simulink model "CombinedExperiment"  (R2020a)
settings: Solver=FixedStepAuto  StartTime=0.0  StopTime=tsim  FixedStep=baseRate  RelTol=1e-3  EnableMultiTasking=on
values from neighbouring files (symbols this model uses):
  baseRate = 0.1    [Run_Initializer.m]
  drop_states_BLACK = [1.36947387695313,1.22175756835938,-0.0161599479615688]    [Run_Initializer.m]
  drop_states_BLUE = [ xLength/2+0.9; yLength/2+0.5; 0]    [Run_Initializer.m]
  drop_states_RED = [ xLength/2+1.1; yLength/2; pi]    [Run_Initializer.m]
  F_thrusters_BLACK = 0.25.*ones(8,1)    [Run_Initializer.m]
  F_thrusters_BLUE = 0.25.*ones(8,1)    [Run_Initializer.m]
  F_thrusters_RED = 0.25.*ones(8,1)    [Run_Initializer.m]
  home_states_BLACK = [ xLength/2; yLength/2; 0]    [Run_Initializer.m]
  home_states_BLUE = [ xLength/2-0.9; yLength/2+0.5; 0]    [Run_Initializer.m]
  home_states_RED = [ xLength/2+1.1; yLength/2; pi]    [Run_Initializer.m]
  init_states_BLACK = [ xLength/2; yLength/2; 0]    [Run_Initializer.m]
  init_states_BLUE = [ xLength/2+0.9; yLength/2+0.5; 0]    [Run_Initializer.m]
  init_states_RED = [ xLength/2+1.1; yLength/2; pi]    [Run_Initializer.m]
  Kd_tb = 0.4    [Run_Initializer.m]
  Kd_tblue = 0.4    [Run_Initializer.m]
  Kd_tr = 0.4    [Run_Initializer.m]
  Kd_xb = 5    [Run_Initializer.m]
  Kd_xblue = 5    [Run_Initializer.m]
  Kd_xr = 5    [Run_Initializer.m]
  Kd_yb = 5    [Run_Initializer.m]
  Kd_yblue = 5    [Run_Initializer.m]
  Kd_yr = 5    [Run_Initializer.m]
  Kp_tb = 0.1    [Run_Initializer.m]
  Kp_tblue = 0.1    [Run_Initializer.m]
  Kp_tr = 0.1    [Run_Initializer.m]
  Kp_xb = 2    [Run_Initializer.m]
  Kp_xblue = 2    [Run_Initializer.m]
  Kp_xr = 2    [Run_Initializer.m]
  Kp_yb = 2    [Run_Initializer.m]
  Kp_yblue = 2    [Run_Initializer.m]
  Kp_yr = 2    [Run_Initializer.m]
  noise_variance_BLACK = 0    [Run_Initializer.m]
  noise_variance_BLUE = 0    [Run_Initializer.m]
  noise_variance_RED = 0    [Run_Initializer.m]
  Phase0_End = Phase0_Duration    (= 10)    [Run_Initializer.m]
  Phase1_End = Phase0_Duration + Phase1_Duration    (= 15)    [Run_Initializer.m]
  Phase2_End = Phase0_Duration + Phase1_Duration +                                   Phase2_Duration    (= 40)    [Run_Initializer.m]
  Phase3_End = Phase0_Duration + Phase1_Duration +                                   Phase2_Duration + Phase3_Duration    (= 117)    [Run_Initializer.m]
  Phase3_SubPhase1_End = Phase2_End + Phase3_SubPhase1_Duration    (= 41)    [Run_Initializer.m]
  Phase3_SubPhase2_End = Phase2_End + Phase3_SubPhase1_Duration +                                   Phase3_SubPhase2_Duration    (= 42)    [Run_Initializer.m]
  Phase3_SubPhase3_End = Phase2_End + Phase3_SubPhase1_Duration +                                   Phase3_SubPhase2_Duration +                                  Phase3_SubPhase3_Duration    (= 72)    [Run_Initializer.m]
  Phase3_SubPhase4_End = Phase2_End + Phase3_SubPhase1_Duration +                                   Phase3_SubPhase2_Duration +                                  Phase3_SubPhase3_Duration +                                  Phase3_SubPhase4_Duration    [Run_Initializer.m]
  Phase4_End = Phase0_Duration + Phase1_Duration +                                   Phase2_Duration + Phase3_Duration +                                   Phase4_Duration    (= 137)    [Run_Initializer.m]
  Phase5_End = Phase0_Duration + Phase1_Duration +                                   Phase2_Duration + Phase3_Duration +                                   Phase4_Duration + Phase5_Duration    (= 142)    [Run_Initializer.m]
  serverRate = 0.2    [Run_Initializer.m]
  thruster_dist2CG_BLACK = [83.42;-52.58;55.94;-60.05;54.08;-53.92;77.06;-55.94]    [Run_Initializer.m]
  thruster_dist2CG_BLUE = [83.42;-52.58;55.94;-60.05;54.08;-53.92;77.06;-55.94]    [Run_Initializer.m]
  thruster_dist2CG_RED = [49.92;-78.08;70.46;-63.54;81.08;-50.42;57.44;-75.96]    [Run_Initializer.m]
  xLength = 3.51155    [Run_Initializer.m]
  yLength = 2.41935    [Run_Initializer.m]
undefined symbols (not defined in the file or in its folder): DiscIntNeverNeededParam, platformSelection, simMode, WhoAmI
libraries: dspstat3 x18, raspberrypiBasiclib x10, dspsigops x9, embdlinuxlib x8, simulink x8, MainLibrary x5, mspfiltlib x3, dsparch4 x3, dspswit3 x2, sensehatlib x1
(part 3 of 9)

== system CombinedExperiment/Phase #2: Move to Initial Position/Change BLACK Behavior ==
  note: Additional Blocks
  note: PD Control Law - BLACK
  note: Additional blocks are stored here.
  note: A simple PD control law is used here to command the platform to it's initial position, as defined in the initializer.
  Action Port : ActionPort  ActionPortLabel=if(u1 == 2 | u2 == 1)
  BLACK_Fx : DataStoreWrite  DataStoreName=BLACK_Fx
  BLACK_Fy : DataStoreWrite  DataStoreName=BLACK_Fy
  BLACK_Px : DataStoreRead  DataStoreName=BLACK_Px
  "BLACK_Py " : DataStoreRead  DataStoreName=BLACK_Py
  BLACK_Rz : DataStoreRead  DataStoreName=BLACK_Rz
  BLACK_Tz : DataStoreWrite  DataStoreName=BLACK_Tz
  Custom Discrete PD (Attitude) : Subsystem
  Custom Discrete PD (X-Position) : Subsystem
  Custom Discrete PD (Y-Position) : Subsystem
  Data Store Write3 : DataStoreWrite  DataStoreName=Float_State
  Desired Attitude (BLACK) : Constant  Value=init_states_BLACK(3)  SampleTime=-1
  Desired Px (BLACK) : Constant  Value=init_states_BLACK(1)  SampleTime=-1
  Desired Py (BLACK) : Constant  Value=init_states_BLACK(2)  SampleTime=-1
  Hough Control : Subsystem
  Puck State : Constant
  Subtract : Sum  Inputs=+-
  Subtract1 : Sum  Inputs=+-
  wires:
  Custom Discrete PD (Y-Position)/1(Fy) -> BLACK_Fy/1
  Hough Control/1(Err) -> Custom Discrete PD (Attitude)/1(ez)
  BLACK_Px/1 -> Subtract/2
  Subtract1/1 -> Custom Discrete PD (Y-Position)/1(ey)
  Custom Discrete PD (Attitude)/1(Tz) -> BLACK_Tz/1
  "BLACK_Py "/1 -> Subtract1/2
  Subtract/1 -> Custom Discrete PD (X-Position)/1(ex)
  Custom Discrete PD (X-Position)/1(Fx) -> BLACK_Fx/1
  Desired Px (BLACK)/1 -> Subtract/1
  Desired Py (BLACK)/1 -> Subtract1/1
  Desired Attitude (BLACK)/1 -> Hough Control/1(Ref)
  BLACK_Rz/1 -> Hough Control/2(Act)
  Puck State/1 -> Data Store Write3/1

== system CombinedExperiment/Phase #2: Move to Initial Position/Change BLUE Behavior ==
  note: PD Control Law - BLUE
  note: Additional blocks are stored here.
  note: A simple PD control law is used here to command the platform to it's initial position, as defined in the initializer.
  note: Additional Blocks
  Action Port : ActionPort  ActionPortLabel=if(u1 == 3 | u2 == 1)
  BLUE_Fx : DataStoreWrite  DataStoreName=BLUE_Fx
  BLUE_Fy : DataStoreWrite  DataStoreName=BLUE_Fy
  BLUE_Px : DataStoreRead  DataStoreName=BLUE_Px
  "BLUE_Py " : DataStoreRead  DataStoreName=BLUE_Py
  BLUE_Rz : DataStoreRead  DataStoreName=BLUE_Rz
  BLUE_Tz : DataStoreWrite  DataStoreName=BLUE_Tz
  Custom Discrete PD (Attitude) : Subsystem
  Custom Discrete PD (X-Position) : Subsystem
  Custom Discrete PD (Y-Position) : Subsystem
  Data Store Write3 : DataStoreWrite  DataStoreName=Float_State
  Desired Attitude (BLUE) : Constant  Value=init_states_BLUE(3)  SampleTime=-1
  Desired Px (BLUE) : Constant  Value=init_states_BLUE(1)  SampleTime=-1
  Desired Py (BLUE) : Constant  Value=init_states_BLUE(2)  SampleTime=-1
  Hough Control : Subsystem
  Puck State : Constant
  Subtract : Sum  Inputs=+-
  Subtract1 : Sum  Inputs=+-
  wires:
  Desired Attitude (BLUE)/1 -> Hough Control/1(Ref)
  BLUE_Rz/1 -> Hough Control/2(Act)
  Puck State/1 -> Data Store Write3/1
  Subtract/1 -> Custom Discrete PD (X-Position)/1(ex)
  Hough Control/1(Err) -> Custom Discrete PD (Attitude)/1(ez)
  Custom Discrete PD (X-Position)/1(Fx) -> BLUE_Fx/1
  Desired Py (BLUE)/1 -> Subtract1/1
  BLUE_Px/1 -> Subtract/2
  Subtract1/1 -> Custom Discrete PD (Y-Position)/1(ey)
  Desired Px (BLUE)/1 -> Subtract/1
  "BLUE_Py "/1 -> Subtract1/2
  Custom Discrete PD (Y-Position)/1(Fy) -> BLUE_Fy/1
  Custom Discrete PD (Attitude)/1(Tz) -> BLUE_Tz/1

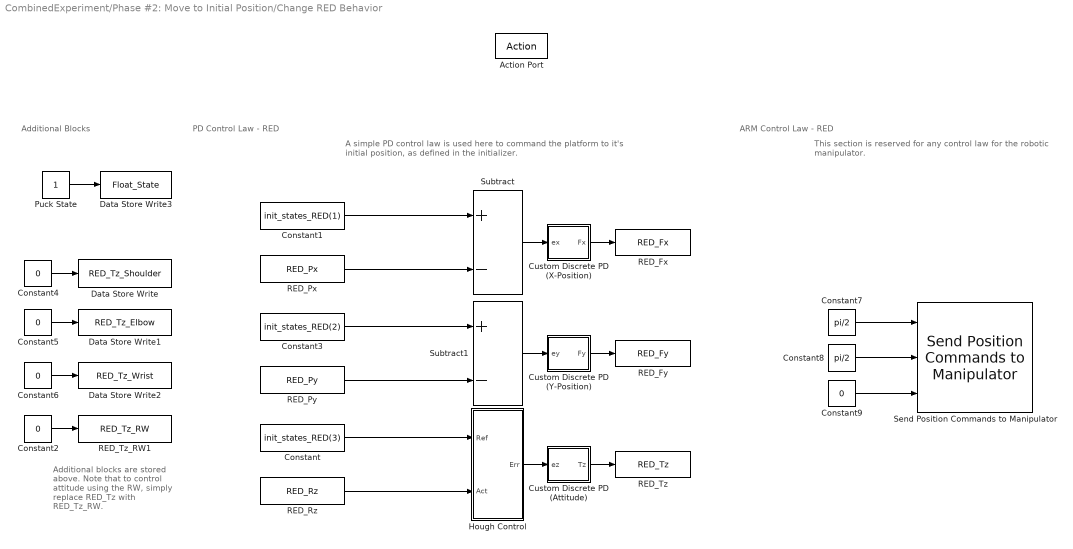
== system CombinedExperiment/Phase #2: Move to Initial Position/Change RED Behavior ==
  note: ARM Control Law - RED
  note: PD Control Law - RED
  note: Additional Blocks
  note: Additional blocks are stored above. Note that to control attitude using the RW, simply replace RED_Tz with RED_Tz_RW.
  note: A simple PD control law is used here to command the platform to it's initial position, as defined in the initializer.
  note: This section is reserved for any control law for the robotic manipulator.
  Action Port : ActionPort  ActionPortLabel=if(u1 == 1 | u2 == 1)
  Constant : Constant  Value=init_states_RED(3)
  Constant1 : Constant  Value=init_states_RED(1)
  Constant{2,4..6,9} (5 alike) : Constant  Value=0
  Constant3 : Constant  Value=init_states_RED(2)
  Constant7 : Constant  Value=pi/2
  Constant8 : Constant  Value=pi/2
  Custom Discrete PD (Attitude) : Subsystem
  Custom Discrete PD (X-Position) : Subsystem
  Custom Discrete PD (Y-Position) : Subsystem
  Data Store Write : DataStoreWrite  DataStoreName=RED_Tz_Shoulder
  Data Store Write1 : DataStoreWrite  DataStoreName=RED_Tz_Elbow
  Data Store Write2 : DataStoreWrite  DataStoreName=RED_Tz_Wrist
  Data Store Write3 : DataStoreWrite  DataStoreName=Float_State
  Hough Control : Subsystem
  Puck State : Constant
  RED_Fx : DataStoreWrite  DataStoreName=RED_Fx
  RED_Fy : DataStoreWrite  DataStoreName=RED_Fy
  RED_Px : DataStoreRead  DataStoreName=RED_Px
  "RED_Py " : DataStoreRead  DataStoreName=RED_Py
  RED_Rz : DataStoreRead  DataStoreName=RED_Rz
  RED_Tz : DataStoreWrite  DataStoreName=RED_Tz
  RED_Tz_RW1 : DataStoreWrite  DataStoreName=RED_Tz_RW
  Send Position Commands to Manipulator : MainLibrary/Dynamixel Functions/Send Position Commands to Manipulator
      settings: SourceProductName=SPOT Custom Library
  Subtract : Sum  Inputs=+-
  Subtract1 : Sum  Inputs=+-
  wires:
  Constant6/1 -> Data Store Write2/1
  Constant5/1 -> Data Store Write1/1
  Constant2/1 -> RED_Tz_RW1/1
  Constant4/1 -> Data Store Write/1
  Custom Discrete PD (Attitude)/1(Tz) -> RED_Tz/1
  RED_Rz/1 -> Hough Control/2(Act)
  Custom Discrete PD (X-Position)/1(Fx) -> RED_Fx/1
  Subtract/1 -> Custom Discrete PD (X-Position)/1(ex)
  Hough Control/1(Err) -> Custom Discrete PD (Attitude)/1(ez)
  Custom Discrete PD (Y-Position)/1(Fy) -> RED_Fy/1
  RED_Px/1 -> Subtract/2
  "RED_Py "/1 -> Subtract1/2
  Subtract1/1 -> Custom Discrete PD (Y-Position)/1(ey)
  Constant1/1 -> Subtract/1
  Constant3/1 -> Subtract1/1
  Constant/1 -> Hough Control/1(Ref)
  Puck State/1 -> Data Store Write3/1
  Constant7/1 -> Send Position Commands to Manipulator/1
  Constant8/1 -> Send Position Commands to Manipulator/2
  Constant9/1 -> Send Position Commands to Manipulator/3

== system CombinedExperiment/Phase #2: Move to Initial Position/Is this a simulation? ==
  Constant : Constant  Value=simMode  SampleTime=-1
  isSim : Outport  VectorParamsAs1DForOutWhenUnconnected=off
  wires:
  Constant/1 -> isSim/1

== system CombinedExperiment/Phase #3: Experiment/Change BLACK Behavior ==
  note: For experiments, it is usually desirable to have various sub-phases. The sub-phases are defined in the initializer; note that in the template only three sub-phases are present, but more can be added.
  Action Port : ActionPort  ActionPortLabel=if(u1 == 2 | u2 == 1)
  Constant1 : Constant  Value=Phase3_SubPhase2_End  SampleTime=-1
  Constant2 : Constant  Value=Phase3_SubPhase3_End  SampleTime=-1
  Constant3 : Constant  Value=Phase3_SubPhase4_End  SampleTime=-1
  Constant4 : Constant  Value=Phase3_SubPhase1_End  SampleTime=-1
  Experiment Sub-Phases : If  NumInputs=5  IfExpression=u1 < u2  ElseIfExpressions=u1 < u3, u1 < u4, u1 < u5  ShowElse=off
  Sub-Phase #1 : Subsystem  TreatAsAtomicUnit=on
  "Sub-Phase #2 " : Subsystem  TreatAsAtomicUnit=on
  "Sub-Phase #3 " : Subsystem  TreatAsAtomicUnit=on
  Sub-Phase #4 : Subsystem  TreatAsAtomicUnit=on
  Subsystem : Subsystem
  wires:
  Experiment Sub-Phases/2 -> "Sub-Phase #2 "/Action
  Experiment Sub-Phases/1 -> Sub-Phase #1/Action
  Experiment Sub-Phases/3 -> "Sub-Phase #3 "/Action
  Constant1/1 -> Experiment Sub-Phases/3
  Constant2/1 -> Experiment Sub-Phases/4
  Constant4/1 -> Experiment Sub-Phases/2
  Subsystem/1(Time) -> Experiment Sub-Phases/1
  Constant3/1 -> Experiment Sub-Phases/5
  Experiment Sub-Phases/4 -> Sub-Phase #4/Action

== system CombinedExperiment/Phase #3: Experiment/Change BLUE Behavior ==
  Action Port : ActionPort  ActionPortLabel=if(u1 == 3 | u2 == 1)
  Constant1 : Constant  Value=Phase3_SubPhase2_End  SampleTime=-1
  Constant2 : Constant  Value=Phase3_SubPhase3_End  SampleTime=-1
  Constant3 : Constant  Value=Phase3_SubPhase4_End  SampleTime=-1
  Constant4 : Constant  Value=Phase3_SubPhase1_End  SampleTime=-1
  Experiment Sub-Phases : If  NumInputs=5  IfExpression=u1 < u2  ElseIfExpressions=u1 < u3, u1 < u4, u1 < u5  ShowElse=off
  Sub-Phase #1 : Subsystem  TreatAsAtomicUnit=on
  "Sub-Phase #2 " : Subsystem  TreatAsAtomicUnit=on
  "Sub-Phase #3 " : Subsystem  TreatAsAtomicUnit=on
  Sub-Phase #4 : Subsystem  TreatAsAtomicUnit=on
  Subsystem : Subsystem
  wires:
  Constant3/1 -> Experiment Sub-Phases/5
  Experiment Sub-Phases/4 -> Sub-Phase #4/Action
  Subsystem/1(Time) -> Experiment Sub-Phases/1
  Experiment Sub-Phases/1 -> Sub-Phase #1/Action
  Constant2/1 -> Experiment Sub-Phases/4
  Constant4/1 -> Experiment Sub-Phases/2
  Constant1/1 -> Experiment Sub-Phases/3
  Experiment Sub-Phases/3 -> "Sub-Phase #3 "/Action
  Experiment Sub-Phases/2 -> "Sub-Phase #2 "/Action

== system CombinedExperiment/Phase #3: Experiment/Change RED Behavior ==
  note: For experiments, it is usually desirable to have various sub-phases. The sub-phases are defined in the initializer; note that in the template only three sub-phases are present, but more can be added.
  Action Port : ActionPort  ActionPortLabel=if(u1 == 1 | u2 == 1)
  Constant1 : Constant  Value=Phase3_SubPhase2_End  SampleTime=-1
  Constant2 : Constant  Value=Phase3_SubPhase3_End  SampleTime=-1
  Constant3 : Constant  Value=Phase3_SubPhase4_End  SampleTime=-1
  Constant4 : Constant  Value=Phase3_SubPhase1_End  SampleTime=-1
  Experiment Sub-Phases : If  NumInputs=5  IfExpression=u1 < u2  ElseIfExpressions=u1 < u3, u1 < u4, u1 < u5  ShowElse=off
  Sub-Phase #1 : Subsystem  TreatAsAtomicUnit=on
  "Sub-Phase #2 " : Subsystem  TreatAsAtomicUnit=on
  "Sub-Phase #3 " : Subsystem  TreatAsAtomicUnit=on
  Sub-Phase #4 : Subsystem  TreatAsAtomicUnit=on
  Subsystem : Subsystem
  wires:
  Experiment Sub-Phases/1 -> Sub-Phase #1/Action
  Experiment Sub-Phases/2 -> "Sub-Phase #2 "/Action
  Subsystem/1(Time) -> Experiment Sub-Phases/1
  Experiment Sub-Phases/3 -> "Sub-Phase #3 "/Action
  Constant4/1 -> Experiment Sub-Phases/2
  Constant1/1 -> Experiment Sub-Phases/3
  Constant2/1 -> Experiment Sub-Phases/4
  Constant3/1 -> Experiment Sub-Phases/5
  Experiment Sub-Phases/4 -> Sub-Phase #4/Action

== system CombinedExperiment/Phase #3: Experiment/Is this a simulation? ==
  Constant : Constant  Value=simMode  SampleTime=-1
  isSim : Outport  VectorParamsAs1DForOutWhenUnconnected=off
  wires:
  Constant/1 -> isSim/1

== system CombinedExperiment/Phase #4: Return Home/Change BLACK Behavior ==
  note: Additional Blocks
  note: PD Control Law - BLACK
  note: Additional blocks are stored here.
  note: A simple PD control law is used here to command the platform to it's initial position, as defined in the initializer.
  Action Port : ActionPort  ActionPortLabel=if(u1 == 2 | u2 == 1)
  BLACK_Fx : DataStoreWrite  DataStoreName=BLACK_Fx
  BLACK_Fy : DataStoreWrite  DataStoreName=BLACK_Fy
  BLACK_Px : DataStoreRead  DataStoreName=BLACK_Px
  "BLACK_Py " : DataStoreRead  DataStoreName=BLACK_Py
  BLACK_Rz : DataStoreRead  DataStoreName=BLACK_Rz
  BLACK_Tz : DataStoreWrite  DataStoreName=BLACK_Tz
  Custom Discrete PD (Attitude) : Subsystem
  Custom Discrete PD (X-Position) : Subsystem
  Custom Discrete PD (Y-Position) : Subsystem
  Data Store Write3 : DataStoreWrite  DataStoreName=Float_State
  Desired Attitude (BLACK) : Constant  Value=home_states_BLACK(3)  SampleTime=-1
  Desired Px (BLACK) : Constant  Value=home_states_BLACK(1)  SampleTime=-1
  Desired Py (BLACK) : Constant  Value=home_states_BLACK(2)  SampleTime=-1
  Hough Control : Subsystem
  Puck State : Constant
  Subtract : Sum  Inputs=+-
  Subtract1 : Sum  Inputs=+-
  wires:
  Custom Discrete PD (Y-Position)/1(Fy) -> BLACK_Fy/1
  Desired Py (BLACK)/1 -> Subtract1/1
  Hough Control/1(Err) -> Custom Discrete PD (Attitude)/1(ez)
  BLACK_Px/1 -> Subtract/2
  Subtract1/1 -> Custom Discrete PD (Y-Position)/1(ey)
  Custom Discrete PD (Attitude)/1(Tz) -> BLACK_Tz/1
  Desired Attitude (BLACK)/1 -> Hough Control/1(Ref)
  "BLACK_Py "/1 -> Subtract1/2
  Subtract/1 -> Custom Discrete PD (X-Position)/1(ex)
  BLACK_Rz/1 -> Hough Control/2(Act)
  Desired Px (BLACK)/1 -> Subtract/1
  Custom Discrete PD (X-Position)/1(Fx) -> BLACK_Fx/1
  Puck State/1 -> Data Store Write3/1

== system CombinedExperiment/Phase #4: Return Home/Change BLUE Behavior ==
  note: PD Control Law - BLUE
  note: Additional blocks are stored here.
  note: A simple PD control law is used here to command the platform to it's initial position, as defined in the initializer.
  note: Additional Blocks
  Action Port : ActionPort  ActionPortLabel=if(u1 == 3 | u2 == 1)
  BLUE_Fx : DataStoreWrite  DataStoreName=BLUE_Fx
  BLUE_Fy : DataStoreWrite  DataStoreName=BLUE_Fy
  BLUE_Px : DataStoreRead  DataStoreName=BLUE_Px
  "BLUE_Py " : DataStoreRead  DataStoreName=BLUE_Py
  BLUE_Rz : DataStoreRead  DataStoreName=BLUE_Rz
  BLUE_Tz : DataStoreWrite  DataStoreName=BLUE_Tz
  Custom Discrete PD (Attitude) : Subsystem
  Custom Discrete PD (X-Position) : Subsystem
  Custom Discrete PD (Y-Position) : Subsystem
  Data Store Write3 : DataStoreWrite  DataStoreName=Float_State
  Desired Attitude (BLUE) : Constant  Value=home_states_BLUE(3)  SampleTime=-1
  Desired Px (BLUE) : Constant  Value=home_states_BLUE(1)  SampleTime=-1
  Desired Py (BLUE) : Constant  Value=home_states_BLUE(2)  SampleTime=-1
  Hough Control : Subsystem
  Puck State : Constant
  Subtract : Sum  Inputs=+-
  Subtract1 : Sum  Inputs=+-
  wires:
  Puck State/1 -> Data Store Write3/1
  Subtract/1 -> Custom Discrete PD (X-Position)/1(ex)
  Desired Py (BLUE)/1 -> Subtract1/1
  Custom Discrete PD (X-Position)/1(Fx) -> BLUE_Fx/1
  Desired Px (BLUE)/1 -> Subtract/1
  Subtract1/1 -> Custom Discrete PD (Y-Position)/1(ey)
  Hough Control/1(Err) -> Custom Discrete PD (Attitude)/1(ez)
  Desired Attitude (BLUE)/1 -> Hough Control/1(Ref)
  Custom Discrete PD (Attitude)/1(Tz) -> BLUE_Tz/1
  "BLUE_Py "/1 -> Subtract1/2
  Custom Discrete PD (Y-Position)/1(Fy) -> BLUE_Fy/1
  BLUE_Px/1 -> Subtract/2
  BLUE_Rz/1 -> Hough Control/2(Act)

== system CombinedExperiment/Phase #4: Return Home/Change RED Behavior ==
  note: ARM Control Law - RED
  note: PD Control Law - RED
  note: Additional Blocks
  note: Additional blocks are stored above. Note that to control attitude using the RW, simply replace RED_Tz with RED_Tz_RW.
  note: A simple PD control law is used here to command the platform to it's initial position, as defined in the initializer.
  note: This section is reserved for any control law for the robotic manipulator.
  Action Port : ActionPort  ActionPortLabel=if(u1 == 1 | u2 == 1)
  Constant : Constant  Value=home_states_RED(3)
  Constant1 : Constant  Value=home_states_RED(1)
  Constant{2,4..6} (4 alike) : Constant  Value=0
  Constant3 : Constant  Value=home_states_RED(2)
  Custom Discrete PD (Attitude) : Subsystem
  Custom Discrete PD (X-Position) : Subsystem
  Custom Discrete PD (Y-Position) : Subsystem
  Data Store Write : DataStoreWrite  DataStoreName=RED_Tz_Shoulder
  Data Store Write1 : DataStoreWrite  DataStoreName=RED_Tz_Elbow
  Data Store Write2 : DataStoreWrite  DataStoreName=RED_Tz_Wrist
  Data Store Write3 : DataStoreWrite  DataStoreName=Float_State
  Hough Control : Subsystem
  Puck State : Constant
  RED_Fx : DataStoreWrite  DataStoreName=RED_Fx
  RED_Fy : DataStoreWrite  DataStoreName=RED_Fy
  RED_Px : DataStoreRead  DataStoreName=RED_Px
  "RED_Py " : DataStoreRead  DataStoreName=RED_Py
  RED_Rz : DataStoreRead  DataStoreName=RED_Rz
  RED_Tz : DataStoreWrite  DataStoreName=RED_Tz
  RED_Tz_RW1 : DataStoreWrite  DataStoreName=RED_Tz_RW
  Subtract : Sum  Inputs=+-
  Subtract1 : Sum  Inputs=+-
  wires:
  Constant6/1 -> Data Store Write2/1
  Constant5/1 -> Data Store Write1/1
  Constant2/1 -> RED_Tz_RW1/1
  Constant4/1 -> Data Store Write/1
  Constant1/1 -> Subtract/1
  Custom Discrete PD (Attitude)/1(Tz) -> RED_Tz/1
  Constant/1 -> Hough Control/1(Ref)
  RED_Rz/1 -> Hough Control/2(Act)
  Constant3/1 -> Subtract1/1
  Custom Discrete PD (X-Position)/1(Fx) -> RED_Fx/1
  Subtract/1 -> Custom Discrete PD (X-Position)/1(ex)
  Hough Control/1(Err) -> Custom Discrete PD (Attitude)/1(ez)
  Custom Discrete PD (Y-Position)/1(Fy) -> RED_Fy/1
  RED_Px/1 -> Subtract/2
  "RED_Py "/1 -> Subtract1/2
  Subtract1/1 -> Custom Discrete PD (Y-Position)/1(ey)
  Puck State/1 -> Data Store Write3/1

== system CombinedExperiment/Phase #4: Return Home/Is this a simulation? ==
  Constant : Constant  Value=simMode  SampleTime=-1
  isSim : Outport  VectorParamsAs1DForOutWhenUnconnected=off
  wires:
  Constant/1 -> isSim/1

== system CombinedExperiment/Phase #5: Hold Home/Change BLACK Behavior ==
  note: Additional Blocks
  note: PD Control Law - BLACK
  note: A simple PD control law is used here to command the platform to it's initial position, as defined in the initializer.
  note: Additional blocks are stored here.
  Action Port : ActionPort  ActionPortLabel=if(u1 == 2 | u2 == 1)
  BLACK_Fx : DataStoreWrite  DataStoreName=BLACK_Fx
  BLACK_Fy : DataStoreWrite  DataStoreName=BLACK_Fy
  BLACK_Px : DataStoreRead  DataStoreName=BLACK_Px
  "BLACK_Py " : DataStoreRead  DataStoreName=BLACK_Py
  BLACK_Rz : DataStoreRead  DataStoreName=BLACK_Rz
  BLACK_Tz : DataStoreWrite  DataStoreName=BLACK_Tz
  Constant : Constant  Value=home_states_BLACK(1)
  Constant2 : Constant  Value=home_states_BLACK(2)
  Constant3 : Constant  Value=home_states_BLACK(3)
  Custom Discrete PD (Attitude) : Subsystem
  Custom Discrete PD (X-Position) : Subsystem
  Custom Discrete PD (Y-Position) : Subsystem
  Data Store Write3 : DataStoreWrite  DataStoreName=Float_State
  Hough Control : Subsystem
  Puck State : Constant
  Subtract : Sum  Inputs=+-
  Subtract1 : Sum  Inputs=+-
  wires:
  Custom Discrete PD (X-Position)/1(Fx) -> BLACK_Fx/1
  "BLACK_Py "/1 -> Subtract1/2
  Subtract1/1 -> Custom Discrete PD (Y-Position)/1(ey)
  Custom Discrete PD (Y-Position)/1(Fy) -> BLACK_Fy/1
  Constant3/1 -> Hough Control/1(Ref)
  Constant/1 -> Subtract/1
  Constant2/1 -> Subtract1/1
  Subtract/1 -> Custom Discrete PD (X-Position)/1(ex)
  Hough Control/1(Err) -> Custom Discrete PD (Attitude)/1(ez)
  Custom Discrete PD (Attitude)/1(Tz) -> BLACK_Tz/1
  BLACK_Px/1 -> Subtract/2
  BLACK_Rz/1 -> Hough Control/2(Act)
  Puck State/1 -> Data Store Write3/1

== system CombinedExperiment/Phase #5: Hold Home/Change BLUE Behavior ==
  note: PD Control Law - WHITE
  note: Additional blocks are stored here.
  note: A simple PD control law is used here to command the platform to it's initial position, as defined in the initializer.
  note: Additional Blocks
  Action Port : ActionPort  ActionPortLabel=if(u1 == 3 | u2 == 1)
  BLUE_Fx : DataStoreWrite  DataStoreName=BLUE_Fx
  BLUE_Fy : DataStoreWrite  DataStoreName=BLUE_Fy
  BLUE_Px : DataStoreRead  DataStoreName=BLUE_Px
  "BLUE_Py " : DataStoreRead  DataStoreName=BLUE_Py
  BLUE_Rz : DataStoreRead  DataStoreName=BLUE_Rz
  BLUE_Tz : DataStoreWrite  DataStoreName=BLUE_Tz
  Custom Discrete PD (Attitude) : Subsystem
  Custom Discrete PD (X-Position) : Subsystem
  Custom Discrete PD (Y-Position) : Subsystem
  Data Store Write3 : DataStoreWrite  DataStoreName=Float_State
  Desired Attitude (BLUE) : Constant  Value=home_states_BLUE(3)  SampleTime=-1
  Desired Px (BLUE) : Constant  Value=home_states_BLUE(1)  SampleTime=-1
  Desired Py (BLUE) : Constant  Value=home_states_BLUE(2)  SampleTime=-1
  Hough Control : Subsystem
  Puck State : Constant
  Subtract : Sum  Inputs=+-
  Subtract1 : Sum  Inputs=+-
  wires:
  Puck State/1 -> Data Store Write3/1
  Custom Discrete PD (Y-Position)/1(Fy) -> BLUE_Fy/1
  Custom Discrete PD (X-Position)/1(Fx) -> BLUE_Fx/1
  Subtract1/1 -> Custom Discrete PD (Y-Position)/1(ey)
  "BLUE_Py "/1 -> Subtract1/2
  Desired Px (BLUE)/1 -> Subtract/1
  Hough Control/1(Err) -> Custom Discrete PD (Attitude)/1(ez)
  Subtract/1 -> Custom Discrete PD (X-Position)/1(ex)
  Custom Discrete PD (Attitude)/1(Tz) -> BLUE_Tz/1
  BLUE_Rz/1 -> Hough Control/2(Act)
  Desired Py (BLUE)/1 -> Subtract1/1
  BLUE_Px/1 -> Subtract/2
  Desired Attitude (BLUE)/1 -> Hough Control/1(Ref)

== system CombinedExperiment/Phase #5: Hold Home/Change RED Behavior ==
  note: PD Control Law - RED
  note: ARM Control Law - RED
  note: Additional Blocks
  note: Additional blocks are stored above. Note that to control attitude using the RW, simply replace RED_Tz with RED_Tz_RW.
  note: A simple PD control law is used here to command the platform to it's home position, as defined in the initializer.
  note: This section is reserved for any control law for the robotic manipulator.
  Action Port : ActionPort  ActionPortLabel=if(u1 == 1 | u2 == 1)
  Constant : Constant  Value=home_states_RED(1)
  Constant{1,4..6} (4 alike) : Constant  Value=0
  Constant2 : Constant  Value=home_states_RED(2)
  Constant3 : Constant  Value=home_states_RED(3)
  Custom Discrete PD (Attitude) : Subsystem
  Custom Discrete PD (X-Position) : Subsystem
  Custom Discrete PD (Y-Position) : Subsystem
  Data Store Write : DataStoreWrite  DataStoreName=RED_Tz_Shoulder
  Data Store Write1 : DataStoreWrite  DataStoreName=RED_Tz_Elbow
  Data Store Write2 : DataStoreWrite  DataStoreName=RED_Tz_Wrist
  Data Store Write3 : DataStoreWrite  DataStoreName=Float_State
  Hough Control : Subsystem
  Puck State : Constant
  RED_Fx : DataStoreWrite  DataStoreName=RED_Fx
  RED_Fy : DataStoreWrite  DataStoreName=RED_Fy
  RED_Px : DataStoreRead  DataStoreName=RED_Px
  "RED_Py " : DataStoreRead  DataStoreName=RED_Py
  RED_Rz : DataStoreRead  DataStoreName=RED_Rz
  RED_Tz : DataStoreWrite  DataStoreName=RED_Tz
  RED_Tz_RW : DataStoreWrite  DataStoreName=RED_Tz_RW
  Subtract : Sum  Inputs=+-
  Subtract1 : Sum  Inputs=+-
  wires:
  Constant1/1 -> RED_Tz_RW/1
  Constant5/1 -> Data Store Write1/1
  Constant4/1 -> Data Store Write/1
  Constant6/1 -> Data Store Write2/1
  "RED_Py "/1 -> Subtract1/2
  Custom Discrete PD (Attitude)/1(Tz) -> RED_Tz/1
  Subtract1/1 -> Custom Discrete PD (Y-Position)/1(ey)
  Hough Control/1(Err) -> Custom Discrete PD (Attitude)/1(ez)
  RED_Px/1 -> Subtract/2
  Custom Discrete PD (X-Position)/1(Fx) -> RED_Fx/1
  Subtract/1 -> Custom Discrete PD (X-Position)/1(ex)
  Custom Discrete PD (Y-Position)/1(Fy) -> RED_Fy/1
  Constant/1 -> Subtract/1
  Constant3/1 -> Hough Control/1(Ref)
  RED_Rz/1 -> Hough Control/2(Act)
  Constant2/1 -> Subtract1/1
  Puck State/1 -> Data Store Write3/1

== system CombinedExperiment/Phase #5: Hold Home/Is this a simulation? ==
  Constant : Constant  Value=simMode  SampleTime=-1
  isSim : Outport  VectorParamsAs1DForOutWhenUnconnected=off
  wires:
  Constant/1 -> isSim/1

== system CombinedExperiment/Phase #6: Stop Floating and Spin Down RW/Change BLACK Behavior ==
  note: At the end of the experiment, the pucks must be turned off.
  note: At the end of the experiment, all thrust and arms movement must cease.
  Action Port : ActionPort  ActionPortLabel=if(u1 == 2 | u2 == 1)
  BLACK_Fx : DataStoreWrite  DataStoreName=BLACK_Fx
  BLACK_Fy : DataStoreWrite  DataStoreName=BLACK_Fy
  BLACK_Tz : DataStoreWrite  DataStoreName=BLACK_Tz
  Constant3 : Constant  Value=0
  Constant4 : Constant  Value=0
  Constant5 : Constant  Value=0
  Data Store Write3 : DataStoreWrite  DataStoreName=Float_State
  Puck State : Constant  Value=0
  wires:
  Constant3/1 -> BLACK_Fx/1
  Constant5/1 -> BLACK_Tz/1
  Constant4/1 -> BLACK_Fy/1
  Puck State/1 -> Data Store Write3/1

== system CombinedExperiment/Phase #6: Stop Floating and Spin Down RW/Change BLUE Behavior ==
  note: Before getting good data, the platforms must NOT be floating. So, float is set to be "off".
  note: For the initialization phase, we do not want any thrust. Thus, all commanded forces are zero.
  Action Port : ActionPort  ActionPortLabel=if(u1 == 3 | u2 == 1)
  BLUE_Fx : DataStoreWrite  DataStoreName=BLUE_Fx
  BLUE_Fy : DataStoreWrite  DataStoreName=BLUE_Fy
  BLUE_Tz : DataStoreWrite  DataStoreName=BLUE_Tz
  Constant3 : Constant  Value=0
  Constant4 : Constant  Value=0
  Constant5 : Constant  Value=0
  Data Store Write4 : DataStoreWrite  DataStoreName=Float_State
  Puck State : Constant  Value=0
  wires:
  Constant3/1 -> BLUE_Fx/1
  Constant5/1 -> BLUE_Tz/1
  Constant4/1 -> BLUE_Fy/1
  Puck State/1 -> Data Store Write4/1

== system CombinedExperiment/Phase #6: Stop Floating and Spin Down RW/Change RED Behavior ==
  note: At the end of the experiment, the pucks must be turned off.
  note: At the end of the experiment, all thrust and arms movement must cease.
  note: Once the platform has settled, the RW must be slowly desaturated (assuming it has been used).
  Action Port : ActionPort  ActionPortLabel=if(u1 == 1 | u2 == 1)
  Constant{,1..2,4..6} (6 alike) : Constant  Value=0
  Data Store Write : DataStoreWrite  DataStoreName=RED_Tz_Shoulder
  Data Store Write1 : DataStoreWrite  DataStoreName=RED_Tz_Elbow
  Data Store Write2 : DataStoreWrite  DataStoreName=RED_Tz_Wrist
  Data Store Write3 : DataStoreWrite  DataStoreName=Float_State
  Gain : Gain  Gain=-1
  Puck State : Constant  Value=0
  RED_Fx : DataStoreWrite  DataStoreName=RED_Fx
  RED_Fy : DataStoreWrite  DataStoreName=RED_Fy
  RED_Tz : DataStoreWrite  DataStoreName=RED_Tz
  RED_Tz_RW : DataStoreWrite  DataStoreName=RED_Tz_RW
  RED_dRz_Speed : DataStoreRead  DataStoreName=RED_dRz_RW_Sat
  Saturation : Saturate  UpperLimit=0.005  LowerLimit=-0.005
  wires:
  Constant/1 -> RED_Fx/1
  Constant6/1 -> Data Store Write2/1
  Constant5/1 -> Data Store Write1/1
  RED_dRz_Speed/1 -> Gain/1
  Constant4/1 -> Data Store Write/1
  Saturation/1 -> RED_Tz_RW/1
  Constant1/1 -> RED_Fy/1
  Gain/1 -> Saturation/1
  Constant2/1 -> RED_Tz/1
  Puck State/1 -> Data Store Write3/1

== system CombinedExperiment/Phase #6: Stop Floating and Spin Down RW/Is this a simulation? ==
  Constant : Constant  Value=simMode  SampleTime=-1
  isSim : Outport  VectorParamsAs1DForOutWhenUnconnected=off
  wires:
  Constant/1 -> isSim/1

== system CombinedExperiment/Simulate Plant Dynamics/BLACK Dynamics Model ==
  control_inputs : Inport
  Acceleration to Velocity : DiscreteIntegrator  SampleTime=-1  ICPrevOutput=DiscIntNeverNeededParam  ICPrevScaledInput=DiscIntNeverNeededParam
  MATLAB Function : MATLAB Function  TreatAsAtomicUnit=on
  Random Number : RandomNumber  Variance=noise_variance_BLACK
  Sum : Sum  Inputs=|++
  Velocity to Position : DiscreteIntegrator  InitialCondition=drop_states_BLACK  SampleTime=-1  ICPrevOutput=DiscIntNeverNeededParam  ICPrevScaledInput=DiscIntNeverNeededParam
  states : Outport  VectorParamsAs1DForOutWhenUnconnected=off
  wires:
  control_inputs/1 -> MATLAB Function/1(control_inputs)
  MATLAB Function/1(x_ddot) -> Acceleration to Velocity/1
  Acceleration to Velocity/1 -> Velocity to Position/1
  Velocity to Position/1 -> Sum/1
  Sum/1 -> states/1
  Random Number/1 -> Sum/2

== system CombinedExperiment/Simulate Plant Dynamics/BLUE  Dynamics Model ==
  control_inputs : Inport
  Acceleration to Velocity : DiscreteIntegrator  SampleTime=-1  ICPrevOutput=DiscIntNeverNeededParam  ICPrevScaledInput=DiscIntNeverNeededParam
  MATLAB Function : MATLAB Function  TreatAsAtomicUnit=on
  Random Number : RandomNumber  Variance=noise_variance_BLUE
  Sum : Sum  Inputs=|++
  Velocity to Position : DiscreteIntegrator  InitialCondition=drop_states_BLUE  SampleTime=-1  ICPrevOutput=DiscIntNeverNeededParam  ICPrevScaledInput=DiscIntNeverNeededParam
  states : Outport  VectorParamsAs1DForOutWhenUnconnected=off
  wires:
  control_inputs/1 -> MATLAB Function/1(control_inputs)
  MATLAB Function/1(x_ddot) -> Acceleration to Velocity/1
  Acceleration to Velocity/1 -> Velocity to Position/1
  Velocity to Position/1 -> Sum/1
  Sum/1 -> states/1
  Random Number/1 -> Sum/2

== system CombinedExperiment/Simulate Plant Dynamics/RED Dynamics Model ==
  control_inputs : Inport
  Acceleration to Velocity : DiscreteIntegrator  SampleTime=-1  ICPrevOutput=DiscIntNeverNeededParam  ICPrevScaledInput=DiscIntNeverNeededParam
  MATLAB Function : MATLAB Function  TreatAsAtomicUnit=on
  Random Number : RandomNumber  Variance=noise_variance_RED
  Sum : Sum  Inputs=|++
  Velocity to Position : DiscreteIntegrator  InitialCondition=drop_states_RED  SampleTime=-1  ICPrevOutput=DiscIntNeverNeededParam  ICPrevScaledInput=DiscIntNeverNeededParam
  states : Outport  VectorParamsAs1DForOutWhenUnconnected=off
  wires:
  control_inputs/1 -> MATLAB Function/1(control_inputs)
  MATLAB Function/1(x_ddot) -> Acceleration to Velocity/1
  Acceleration to Velocity/1 -> Velocity to Position/1
  Velocity to Position/1 -> Sum/1
  Sum/1 -> states/1
  Random Number/1 -> Sum/2

== system CombinedExperiment/Simulate Plant Dynamics/Sample and Hold Data to Match PhaseSpace (BLACK) ==
  states : Inport
  Constant1 : Constant  Value=serverRate
  Data Store Read2 : DataStoreRead  DataStoreName=Univ_Time
  MATLAB Function : MATLAB Function  TreatAsAtomicUnit=on
  Sample and Hold1 : dspsigops/Sample and Hold  trig=Rising edge  initCond=drop_states_BLACK  latchinput=off
  states_hold : Outport  VectorParamsAs1DForOutWhenUnconnected=off
  wires:
  states/1 -> Sample and Hold1/1
  Data Store Read2/1 -> MATLAB Function/1(TIME)
  Constant1/1 -> MATLAB Function/2(SERVER)
  MATLAB Function/1(y) -> Sample and Hold1/Trigger
  Sample and Hold1/1 -> states_hold/1

== system CombinedExperiment/Simulate Plant Dynamics/Sample and Hold Data to Match PhaseSpace (BLUE) ==
  states : Inport
  Constant1 : Constant  Value=serverRate
  Data Store Read2 : DataStoreRead  DataStoreName=Univ_Time
  MATLAB Function : MATLAB Function  TreatAsAtomicUnit=on
  Sample and Hold1 : dspsigops/Sample and Hold  trig=Rising edge  initCond=drop_states_BLUE  latchinput=off
  states_hold : Outport  VectorParamsAs1DForOutWhenUnconnected=off
  wires:
  states/1 -> Sample and Hold1/1
  Data Store Read2/1 -> MATLAB Function/1(TIME)
  Constant1/1 -> MATLAB Function/2(SERVER)
  MATLAB Function/1(y) -> Sample and Hold1/Trigger
  Sample and Hold1/1 -> states_hold/1

== system CombinedExperiment/Simulate Plant Dynamics/Sample and Hold Data to Match PhaseSpace (RED) ==
  states : Inport
  Constant : Constant  Value=serverRate
  Data Store Read1 : DataStoreRead  DataStoreName=Univ_Time
  MATLAB Function : MATLAB Function  TreatAsAtomicUnit=on
  Sample and Hold : dspsigops/Sample and Hold  trig=Rising edge  initCond=drop_states_RED  latchinput=off
  "states_hold " : Outport  VectorParamsAs1DForOutWhenUnconnected=off
  wires:
  Data Store Read1/1 -> MATLAB Function/1(TIME)
  Constant/1 -> MATLAB Function/2(SERVER)
  MATLAB Function/1(y) -> Sample and Hold/Trigger
  Sample and Hold/1 -> "states_hold "/1
  states/1 -> Sample and Hold/1

== system CombinedExperiment/Simulate Plant Dynamics/x_dot -> x1 ==
  note: dy/dt ~= (y2-y1)/deltaT
  y(t) : Inport
  Delay1 : Delay  DelayLength=1  InitialConditionSource=Input port
      settings: InputPortMap=u0,p4
  Hold this value : Subsystem  TreatAsAtomicUnit=on
  Sum6 : Sum  Inputs=-+|
  divide by delta T : Gain  Gain=1/serverRate
  "if we went through a \"step\"" : If  IfExpression=u1 ~= 0  ShowElse=off
  dy(t)/dt : Outport  VectorParamsAs1DForOutWhenUnconnected=off
  wires:
  divide by delta T/1 -> dy(t)/dt/1
  Delay1/1 -> Sum6/1
  "if we went through a \"step\""/1 -> Hold this value/Action
  Hold this value/1(Out1) -> divide by delta T/1
  Sum6/1 -> "if we went through a \"step\""/1, Hold this value/1(In1)
  y(t)/1 -> Sum6/2, Delay1/2, Delay1/1

== system CombinedExperiment/Simulate Plant Dynamics/x_dot -> x10 ==
  note: dy/dt ~= (y2-y1)/deltaT
  y(t) : Inport
  Delay1 : Delay  DelayLength=1  InitialConditionSource=Input port
      settings: InputPortMap=u0,p4
  Hold this value : Subsystem  TreatAsAtomicUnit=on
  Sum6 : Sum  Inputs=-+|
  divide by delta T : Gain  Gain=1/serverRate
  "if we went through a \"step\"" : If  IfExpression=u1 ~= 0  ShowElse=off
  dy(t)/dt : Outport  VectorParamsAs1DForOutWhenUnconnected=off
  wires:
  divide by delta T/1 -> dy(t)/dt/1
  Delay1/1 -> Sum6/1
  "if we went through a \"step\""/1 -> Hold this value/Action
  Hold this value/1(Out1) -> divide by delta T/1
  Sum6/1 -> "if we went through a \"step\""/1, Hold this value/1(In1)
  y(t)/1 -> Sum6/2, Delay1/2, Delay1/1

== system CombinedExperiment/Simulate Plant Dynamics/x_dot -> x11 ==
  note: dy/dt ~= (y2-y1)/deltaT
  y(t) : Inport
  Delay1 : Delay  DelayLength=1  InitialConditionSource=Input port
      settings: InputPortMap=u0,p4
  Hold this value : Subsystem  TreatAsAtomicUnit=on
  Sum6 : Sum  Inputs=-+|
  divide by delta T : Gain  Gain=1/serverRate
  "if we went through a \"step\"" : If  IfExpression=u1 ~= 0  ShowElse=off
  dy(t)/dt : Outport  VectorParamsAs1DForOutWhenUnconnected=off
  wires:
  divide by delta T/1 -> dy(t)/dt/1
  Delay1/1 -> Sum6/1
  "if we went through a \"step\""/1 -> Hold this value/Action
  Hold this value/1(Out1) -> divide by delta T/1
  Sum6/1 -> "if we went through a \"step\""/1, Hold this value/1(In1)
  y(t)/1 -> Sum6/2, Delay1/2, Delay1/1

== system CombinedExperiment/Simulate Plant Dynamics/x_dot -> x13 ==
  note: dy/dt ~= (y2-y1)/deltaT
  y(t) : Inport
  Delay1 : Delay  DelayLength=1  InitialConditionSource=Input port
      settings: InputPortMap=u0,p4
  Hold this value : Subsystem  TreatAsAtomicUnit=on
  Sum6 : Sum  Inputs=-+|
  divide by delta T : Gain  Gain=1/serverRate
  "if we went through a \"step\"" : If  IfExpression=u1 ~= 0  ShowElse=off
  dy(t)/dt : Outport  VectorParamsAs1DForOutWhenUnconnected=off
  wires:
  divide by delta T/1 -> dy(t)/dt/1
  Delay1/1 -> Sum6/1
  "if we went through a \"step\""/1 -> Hold this value/Action
  Hold this value/1(Out1) -> divide by delta T/1
  Sum6/1 -> "if we went through a \"step\""/1, Hold this value/1(In1)
  y(t)/1 -> Sum6/2, Delay1/2, Delay1/1

== system CombinedExperiment/Simulate Plant Dynamics/x_dot -> x14 ==
  note: dy/dt ~= (y2-y1)/deltaT
  y(t) : Inport
  Delay1 : Delay  DelayLength=1  InitialConditionSource=Input port
      settings: InputPortMap=u0,p4
  Hold this value : Subsystem  TreatAsAtomicUnit=on
  Sum6 : Sum  Inputs=-+|
  divide by delta T : Gain  Gain=1/serverRate
  "if we went through a \"step\"" : If  IfExpression=u1 ~= 0  ShowElse=off
  dy(t)/dt : Outport  VectorParamsAs1DForOutWhenUnconnected=off
  wires:
  divide by delta T/1 -> dy(t)/dt/1
  Delay1/1 -> Sum6/1
  "if we went through a \"step\""/1 -> Hold this value/Action
  Hold this value/1(Out1) -> divide by delta T/1
  Sum6/1 -> "if we went through a \"step\""/1, Hold this value/1(In1)
  y(t)/1 -> Sum6/2, Delay1/2, Delay1/1

== system CombinedExperiment/Simulate Plant Dynamics/x_dot -> x16 ==
  note: dy/dt ~= (y2-y1)/deltaT
  y(t) : Inport
  Delay1 : Delay  DelayLength=1  InitialConditionSource=Input port
      settings: InputPortMap=u0,p4
  Hold this value : Subsystem  TreatAsAtomicUnit=on
  Sum6 : Sum  Inputs=-+|
  divide by delta T : Gain  Gain=1/serverRate
  "if we went through a \"step\"" : If  IfExpression=u1 ~= 0  ShowElse=off
  dy(t)/dt : Outport  VectorParamsAs1DForOutWhenUnconnected=off
  wires:
  divide by delta T/1 -> dy(t)/dt/1
  Delay1/1 -> Sum6/1
  "if we went through a \"step\""/1 -> Hold this value/Action
  Hold this value/1(Out1) -> divide by delta T/1
  Sum6/1 -> "if we went through a \"step\""/1, Hold this value/1(In1)
  y(t)/1 -> Sum6/2, Delay1/2, Delay1/1

== system CombinedExperiment/Simulate Plant Dynamics/x_dot -> x17 ==
  note: dy/dt ~= (y2-y1)/deltaT
  y(t) : Inport
  Delay1 : Delay  DelayLength=1  InitialConditionSource=Input port
      settings: InputPortMap=u0,p4
  Hold this value : Subsystem  TreatAsAtomicUnit=on
  Sum6 : Sum  Inputs=-+|
  divide by delta T : Gain  Gain=1/serverRate
  "if we went through a \"step\"" : If  IfExpression=u1 ~= 0  ShowElse=off
  dy(t)/dt : Outport  VectorParamsAs1DForOutWhenUnconnected=off
  wires:
  divide by delta T/1 -> dy(t)/dt/1
  Delay1/1 -> Sum6/1
  "if we went through a \"step\""/1 -> Hold this value/Action
  Hold this value/1(Out1) -> divide by delta T/1
  Sum6/1 -> "if we went through a \"step\""/1, Hold this value/1(In1)
  y(t)/1 -> Sum6/2, Delay1/2, Delay1/1

== system CombinedExperiment/Simulate Plant Dynamics/x_dot -> x2 ==
  note: dy/dt ~= (y2-y1)/deltaT
  y(t) : Inport
  Delay1 : Delay  DelayLength=1  InitialConditionSource=Input port
      settings: InputPortMap=u0,p4
  Hold this value : Subsystem  TreatAsAtomicUnit=on
  Sum6 : Sum  Inputs=-+|
  divide by delta T : Gain  Gain=1/serverRate
  "if we went through a \"step\"" : If  IfExpression=u1 ~= 0  ShowElse=off
  dy(t)/dt : Outport  VectorParamsAs1DForOutWhenUnconnected=off
  wires:
  divide by delta T/1 -> dy(t)/dt/1
  Delay1/1 -> Sum6/1
  "if we went through a \"step\""/1 -> Hold this value/Action
  Hold this value/1(Out1) -> divide by delta T/1
  Sum6/1 -> "if we went through a \"step\""/1, Hold this value/1(In1)
  y(t)/1 -> Sum6/2, Delay1/2, Delay1/1

== system CombinedExperiment/Simulate Plant Dynamics/x_dot -> x3 ==
  note: dy/dt ~= (y2-y1)/deltaT
  y(t) : Inport
  Delay1 : Delay  DelayLength=1  InitialConditionSource=Input port
      settings: InputPortMap=u0,p4
  Hold this value : Subsystem  TreatAsAtomicUnit=on
  Sum6 : Sum  Inputs=-+|
  divide by delta T : Gain  Gain=1/serverRate
  "if we went through a \"step\"" : If  IfExpression=u1 ~= 0  ShowElse=off
  dy(t)/dt : Outport  VectorParamsAs1DForOutWhenUnconnected=off
  wires:
  divide by delta T/1 -> dy(t)/dt/1
  Delay1/1 -> Sum6/1
  "if we went through a \"step\""/1 -> Hold this value/Action
  Hold this value/1(Out1) -> divide by delta T/1
  Sum6/1 -> "if we went through a \"step\""/1, Hold this value/1(In1)
  y(t)/1 -> Sum6/2, Delay1/2, Delay1/1

== system CombinedExperiment/Simulate Plant Dynamics/x_dot -> x4 ==
  note: dy/dt ~= (y2-y1)/deltaT
  y(t) : Inport
  Delay1 : Delay  DelayLength=1  InitialConditionSource=Input port
      settings: InputPortMap=u0,p4
  Hold this value : Subsystem  TreatAsAtomicUnit=on
  Sum6 : Sum  Inputs=-+|
  divide by delta T : Gain  Gain=1/serverRate
  "if we went through a \"step\"" : If  IfExpression=u1 ~= 0  ShowElse=off
  dy(t)/dt : Outport  VectorParamsAs1DForOutWhenUnconnected=off
  wires:
  divide by delta T/1 -> dy(t)/dt/1
  Delay1/1 -> Sum6/1
  "if we went through a \"step\""/1 -> Hold this value/Action
  Hold this value/1(Out1) -> divide by delta T/1
  Sum6/1 -> "if we went through a \"step\""/1, Hold this value/1(In1)
  y(t)/1 -> Sum6/2, Delay1/2, Delay1/1

== system CombinedExperiment/Simulate Plant Dynamics/x_dot -> x5 ==
  note: dy/dt ~= (y2-y1)/deltaT
  y(t) : Inport
  Delay1 : Delay  DelayLength=1  InitialConditionSource=Input port
      settings: InputPortMap=u0,p4
  Hold this value : Subsystem  TreatAsAtomicUnit=on
  Sum6 : Sum  Inputs=-+|
  divide by delta T : Gain  Gain=1/serverRate
  "if we went through a \"step\"" : If  IfExpression=u1 ~= 0  ShowElse=off
  dy(t)/dt : Outport  VectorParamsAs1DForOutWhenUnconnected=off
  wires:
  divide by delta T/1 -> dy(t)/dt/1
  Delay1/1 -> Sum6/1
  "if we went through a \"step\""/1 -> Hold this value/Action
  Hold this value/1(Out1) -> divide by delta T/1
  Sum6/1 -> "if we went through a \"step\""/1, Hold this value/1(In1)
  y(t)/1 -> Sum6/2, Delay1/2, Delay1/1

== system CombinedExperiment/Simulate Plant Dynamics/x_dot -> x6 ==
  note: dy/dt ~= (y2-y1)/deltaT
  y(t) : Inport
  Delay1 : Delay  DelayLength=1  InitialConditionSource=Input port
      settings: InputPortMap=u0,p4
  Hold this value : Subsystem  TreatAsAtomicUnit=on
  Sum6 : Sum  Inputs=-+|
  divide by delta T : Gain  Gain=1/serverRate
  "if we went through a \"step\"" : If  IfExpression=u1 ~= 0  ShowElse=off
  dy(t)/dt : Outport  VectorParamsAs1DForOutWhenUnconnected=off
  wires:
  divide by delta T/1 -> dy(t)/dt/1
  Delay1/1 -> Sum6/1
  "if we went through a \"step\""/1 -> Hold this value/Action
  Hold this value/1(Out1) -> divide by delta T/1
  Sum6/1 -> "if we went through a \"step\""/1, Hold this value/1(In1)
  y(t)/1 -> Sum6/2, Delay1/2, Delay1/1

== system CombinedExperiment/Simulate Plant Dynamics/x_dot -> x7 ==
  note: dy/dt ~= (y2-y1)/deltaT
  y(t) : Inport
  Delay1 : Delay  DelayLength=1  InitialConditionSource=Input port
      settings: InputPortMap=u0,p4
  Hold this value : Subsystem  TreatAsAtomicUnit=on
  Sum6 : Sum  Inputs=-+|
  divide by delta T : Gain  Gain=1/serverRate
  "if we went through a \"step\"" : If  IfExpression=u1 ~= 0  ShowElse=off
  dy(t)/dt : Outport  VectorParamsAs1DForOutWhenUnconnected=off
  wires:
  divide by delta T/1 -> dy(t)/dt/1
  Delay1/1 -> Sum6/1
  "if we went through a \"step\""/1 -> Hold this value/Action
  Hold this value/1(Out1) -> divide by delta T/1
  Sum6/1 -> "if we went through a \"step\""/1, Hold this value/1(In1)
  y(t)/1 -> Sum6/2, Delay1/2, Delay1/1

== system CombinedExperiment/Simulate Plant Dynamics/x_dot -> x8 ==
  note: dy/dt ~= (y2-y1)/deltaT
  y(t) : Inport
  Delay1 : Delay  DelayLength=1  InitialConditionSource=Input port
      settings: InputPortMap=u0,p4
  Hold this value : Subsystem  TreatAsAtomicUnit=on
  Sum6 : Sum  Inputs=-+|
  divide by delta T : Gain  Gain=1/serverRate
  "if we went through a \"step\"" : If  IfExpression=u1 ~= 0  ShowElse=off
  dy(t)/dt : Outport  VectorParamsAs1DForOutWhenUnconnected=off
  wires:
  divide by delta T/1 -> dy(t)/dt/1
  Delay1/1 -> Sum6/1
  "if we went through a \"step\""/1 -> Hold this value/Action
  Hold this value/1(Out1) -> divide by delta T/1
  Sum6/1 -> "if we went through a \"step\""/1, Hold this value/1(In1)
  y(t)/1 -> Sum6/2, Delay1/2, Delay1/1

== system CombinedExperiment/Simulate Plant Dynamics/x_dot -> x9 ==
  note: dy/dt ~= (y2-y1)/deltaT
  y(t) : Inport
  Delay1 : Delay  DelayLength=1  InitialConditionSource=Input port
      settings: InputPortMap=u0,p4
  Hold this value : Subsystem  TreatAsAtomicUnit=on
  Sum6 : Sum  Inputs=-+|
  divide by delta T : Gain  Gain=1/serverRate
  "if we went through a \"step\"" : If  IfExpression=u1 ~= 0  ShowElse=off
  dy(t)/dt : Outport  VectorParamsAs1DForOutWhenUnconnected=off
  wires:
  divide by delta T/1 -> dy(t)/dt/1
  Delay1/1 -> Sum6/1
  "if we went through a \"step\""/1 -> Hold this value/Action
  Hold this value/1(Out1) -> divide by delta T/1
  Sum6/1 -> "if we went through a \"step\""/1, Hold this value/1(In1)
  y(t)/1 -> Sum6/2, Delay1/2, Delay1/1

== system CombinedExperiment/From Force//Torque to PWM Signal/Change BLACK Behavior/Calculate Thruster ON//OFF ==
  note: Calculate which thrusters must be turned on and for how long.
  note: The H matrix is not square, thus a pserudo-inverse is required.
  note: Knowing how much force each thruster can output, we can determine the saturated thruster output and then convert is into a percentage of time over which each thruster is open.
  note: After finding the PWM value, we can use the H matrix to go back to torque and force. However, these torques and forces will be "saturated".
  "[Fx_b; Fy_b; Tz]" : Inport
  BLACK_Fx_Sat : DataStoreWrite  DataStoreName=BLACK_Fx_Sat
  BLACK_Fy_Sat : DataStoreWrite  DataStoreName=BLACK_Fy_Sat
  BLACK_Rz : DataStoreRead  DataStoreName=BLACK_Rz
  BLACK_Tz_Sat : DataStoreWrite  DataStoreName=BLACK_Tz_Sat
  Demux : Demux  Outputs=3
  Demux1 : Demux  Outputs=2
  MATLAB Function : MATLAB Function  TreatAsAtomicUnit=on
  MATLAB Function1 : MATLAB Function  TreatAsAtomicUnit=on
  MATLAB Function2 : MATLAB Function  TreatAsAtomicUnit=on
  Mux : Mux  Inputs=2
  Product : Product  Multiplication=Matrix(*)
  Product1 : Product  Multiplication=Matrix(*)
  Remove Negatives : Saturate  UpperLimit=1000  LowerLimit=0
  Rotate Forces to Inertial : Subsystem
  pseudo-inverse : Subsystem
  ThrusterPWM : Outport  VectorParamsAs1DForOutWhenUnconnected=off
  wires:
  pseudo-inverse/1(invH) -> Product/1
  Product/1 -> Remove Negatives/1
  "[Fx_b; Fy_b; Tz]"/1 -> Product/2
  MATLAB Function/1(H) -> pseudo-inverse/1(H)
  Remove Negatives/1 -> MATLAB Function2/1(ThrustPer)
  MATLAB Function1/1(H) -> Product1/1
  Product1/1 -> Demux/1
  Demux/2 -> Mux/2
  Demux/1 -> Mux/1
  Mux/1 -> Rotate Forces to Inertial/1("F_b ")
  BLACK_Rz/1 -> Rotate Forces to Inertial/2(Rz)
  Demux/3 -> BLACK_Tz_Sat/1
  Rotate Forces to Inertial/1(F_I) -> Demux1/1
  Demux1/1 -> BLACK_Fx_Sat/1
  Demux1/2 -> BLACK_Fy_Sat/1
  MATLAB Function2/1(ThrustPer_Final) -> Product1/2, ThrusterPWM/1

== system CombinedExperiment/From Force//Torque to PWM Signal/Change BLACK Behavior/Rotate Forces to Body ==
  "F_I " : Inport
  Rz : Inport  Port=2
  Create Rotation Matrix : MATLAB Function  TreatAsAtomicUnit=on
  Rotate F_I to F_b : Product  Multiplication=Matrix(*)
  F_b : Outport  VectorParamsAs1DForOutWhenUnconnected=off
  wires:
  Rotate F_I to F_b/1 -> F_b/1
  Create Rotation Matrix/1(C_bI) -> Rotate F_I to F_b/1
  "F_I "/1 -> Rotate F_I to F_b/2
  Rz/1 -> Create Rotation Matrix/1(Rz)
